simulink model "helicopter"  (R2020b)
settings: Solver=ode1  StartTime=0.0  StopTime=simulation_time  FixedStep=0.002  RelTol=1e-3  EnableMultiTasking=on
PostLoadFcn:
  | qc_set_target_type(getConfigSet(bdroot, 'QUARC Default Target Configuration'));
values from neighbouring files (symbols this model uses):
  elevation_gain = 1    [init.m]
  K_ed = 2*d_e*sqrt(K_ep/K_3)    [init.m]
  K_ei = K_ep*0.1    (= 0.348080190282)    [init.m]
  K_ep = w_e^2/K_3    (= 3.48080190282)    [init.m]
  K_pd = 2*d_p*sqrt(K_pp/K_1)    [init.m]
  K_pp = w_p^2/K_1    (= 5.8991559633)    [init.m]
  travel_gain = 1    [init.m]
  Vd_ff = V_d_eq    (= 0.1)    [init.m]
  Vs_ff = V_s_eq    (= 7.88)    [init.m]
  x1_0 = pi    (= 3.14159265359)    [problem_2.m]    (also in problem_4.m)
undefined symbols (not defined in the file or in its folder): HIL, K, qc_get_step_size
libraries: simulink_extras x9, quarc_library x4
settings Model: SimulationMode=external  ExtModeTrigDuration=5000  Creator=Rchan  LastModifiedBy=theodokl
settings SolverCC: PositivePriorityOrder=on
settings DataIOCC: SaveFormat=Array  SignalLoggingSaveFormat=ModelDataLogs  ReturnWorkspaceOutputs=off
settings OptimizationCC: ExpressionDepthLimit=2147483647  InitFltsAndDblsToZero=on  LifeSpan=inf
settings DebuggingCC: SaveWithParameterizedLinksMsg=none  UnderspecifiedInitializationDetection=Classic  MergeDetectMultiDrivingBlocksExec=none  SolverPrmCheckMsg=warning  MultiTaskDSMMsg=warning  MultiTaskCondExecSysMsg=none  FcnCallInpInsideContextMsg=warning  AllowSymbolicDim=off  StateNameClashWarn=warning  SFUnexpectedBacktrackingDiag=warning  SFNoUnconditionalDefaultTransitionDiag=warning  SFExecutionAtInitializationDiag=none  ArithmeticOperatorsInVariantConditions=warning
settings HardwareCC: ProdBitPerPointer=32  ProdBitPerSizeT=32  ProdBitPerPtrDiffT=32  ProdLargestAtomicFloat=None  ProdIntDivRoundTo=Undefined  ProdEndianess=Unspecified  ProdWordSize=32  ProdHWDeviceType=32-bit Generic
settings ModelReferenceCC: PropagateSignalLabelsOutOfModel=off
settings SFSimCC: SimUseLocalCustomCode=off  CustomCodeUndefinedFunction=UseInterfaceOnly
settings RTWCC: Description=QUARC Win64 Target  SystemTargetFile=quarc_win64.tlc  TemplateMakefile=quarc_default_tmf  RTWUseLocalCustomCode=off
settings CodeAppCC: StateflowObjectComments=on
settings GRTTargetCC: TargetLangStandard=C89/C90 (ANSI)  ParMdlRefBuildCompliant=off  CompOptLevelCompliant=off  CombineOutputUpdateFcns=off  MatFileLogging=off  GRTInterface=on  UseToolchainInfoCompliant=off  ExtMode=on  ExtModeMexFile=quarc_comm
settings ConfigComp: CovMetricSettings=dw  CovSaveCumulativeToWorkspaceVar=on  CovSaveSingleToWorkspaceVar=on  CovExternalEMLEnable=off  CovSFcnEnable=off

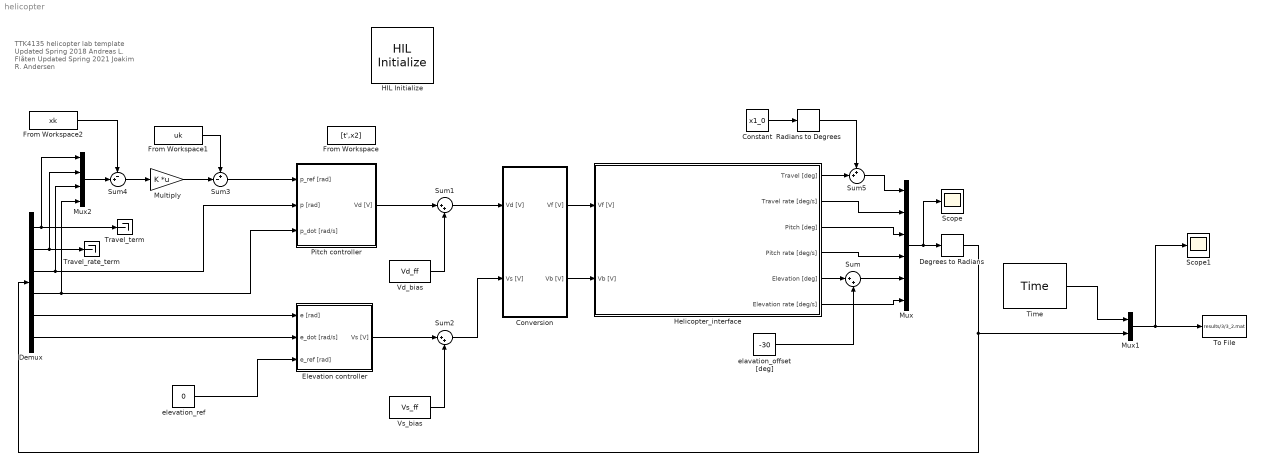
== system helicopter ==
  note: TTK4135 helicopter lab template
      | Updated Spring 2018
      | Andreas L. Flåten
      |
      | Updated Spring 2021
      | Joakim R. Andersen
  Constant : Constant  Value=x1_0
  Conversion : Subsystem
  Degrees to Radians : simulink_extras/Transformations/Degrees to Radians
  Demux : Demux  Outputs=6
  Elevation controller : Subsystem
  From Workspace : FromWorkspace  VariableName=[t',x2]  SampleTime=-1  OutputAfterFinalValue=Holding final value
  From Workspace1 : FromWorkspace  VariableName=uk
  From Workspace2 : FromWorkspace  VariableName=xk
  HIL Initialize : quarc_library/Data Acquisition/Generic/Configuration/HIL Initialize  Priority=-99  object_name=HIL-1  board_type=q8_usb  board_number=0  board_options=update_rate=normal;decimation=1  exclusive=off  active=off  hardware_clocks=[0:2]  clock_modes=[]  initial_clock_frequencies=[]  set_clock_params_at_start=off  set_clock_params_at_switch_in=off  set_clock_frequencies_at_start=off  set_clock_frequencies_at_switch_in=off  analog_input_channels=[0:7]  analog_input_configurations=[]  analog_input_maximums=10  analog_input_minimums=-10  set_analog_input_params_at_start=on  set_analog_input_params_at_switch_in=off  analog_output_channels=[0:7]  analog_output_maximums=10  analog_output_minimums=-10  initial_analog_outputs=[0]  final_analog_outputs=[0]  watchdog_analog_outputs=0  set_analog_output_params_at_start=on  set_analog_output_params_at_switch_in=off  set_analog_outputs_at_start=on  set_analog_outputs_at_switch_in=off  set_analog_outputs_at_terminate=on  set_analog_outputs_at_switch_out=off  set_analog_outputs_on_watchdog=off  digital_input_channels=[]  digital_output_channels=[]  digital_output_configuration=[]  initial_digital_outputs=[1]  final_digital_outputs=[1]  watchdog_digital_outputs=[1]  set_digital_output_params_at_start=off  set_digital_output_params_at_switch_in=off  set_digital_outputs_at_start=on  set_digital_outputs_at_switch_in=off  set_digital_outputs_at_terminate=on  set_digital_outputs_at_switch_out=off  set_digital_outputs_on_watchdog=off  encoder_channels=[0:7]  quadrature=[4]  encoder_filter_frequency=[]  initial_encoder_counts=[0]  set_encoder_params_at_start=on  set_encoder_params_at_switch_in=off  set_encoder_counts_at_start=on  set_encoder_counts_at_switch_in=off  pwm_channels=[0:7]  pwm_modes=0  pwm_frequency=99.532799999999995e6/4095  pwm_configuration=[0]  pwm_alignment=[0]  pwm_polarity=[1]  pwm_leading_deadband=[0]  pwm_trailing_deadband=[0]  initial_pwm_outputs=[0]  final_pwm_outputs=[0]  watchdog_pwm_outputs=[0]  set_pwm_params_at_start=on  set_pwm_params_at_switch_in=off  set_pwm_outputs_at_start=on  set_pwm_outputs_at_switch_in=off  set_pwm_outputs_at_terminate=on  set_pwm_outputs_at_switch_out=off  set_pwm_outputs_on_watchdog=off  other_output_channels=[]  initial_other_outputs=[]  final_other_outputs=[]  watchdog_other_outputs=[]  set_other_outputs_at_start=off  set_other_outputs_at_switch_in=off  set_other_outputs_at_terminate=off  set_other_outputs_at_switch_out=off  set_other_outputs_on_watchdog=off
  Helicopter_interface : Subsystem
  Multiply : Gain  Gain=K  Multiplication=Matrix(K*u)
  Mux : Mux  Inputs=6
  Mux1 : Mux  Inputs=2
  Mux2 : Mux
  Pitch controller : Subsystem
  Radians to Degrees : simulink_extras/Transformations/Radians to Degrees
  Scope : Scope
  Scope1 : Scope
  Sum : Sum  Inputs=|++
  Sum1 : Sum  Inputs=|++
  Sum2 : Sum  Inputs=|++
  Sum3 : Sum  Inputs=+-|
  Sum4 : Sum  Inputs=-+|
  Sum5 : Sum  Inputs=++|
  Time : quarc_library/Sources/Time/Time  time_source=Wall clock  sample_time=qc_get_step_size
  To File : ToFile  Filename=results/3/3_2.mat  MatrixName=simout
  Travel_rate_term : Terminator
  Travel_term : Terminator
  Vd_bias : Constant  Value=Vd_ff
  Vs_bias : Constant  Value=Vs_ff
  elavation_offset [deg] : Constant  Value=-30
  elevation_ref : Constant  Value=0
  wires:
  Conversion/2(Vb [V]) -> Helicopter_interface/2(Vb [V])
  Conversion/1(Vf [V]) -> Helicopter_interface/1(Vf [V])
  elavation_offset [deg]/1 -> Sum/2
  Helicopter_interface/5(Elevation [deg]) -> Sum/1
  Helicopter_interface/4(Pitch rate [deg/s]) -> Mux/4
  Helicopter_interface/3(Pitch [deg]) -> Mux/3
  Helicopter_interface/2(Travel rate [deg/s]) -> Mux/2
  Sum/1 -> Mux/5
  Helicopter_interface/6(Elevation rate [deg/s]) -> Mux/6
  Mux/1 -> Scope/1, Degrees to Radians/1
  Degrees to Radians/1 -> Mux1/2, Demux/1
  Demux/1 -> Mux2/1, Travel_term/1
  Demux/2 -> Mux2/2, Travel_rate_term/1
  Demux/3 -> Mux2/3, Pitch controller/2(p [rad])
  Demux/4 -> Pitch controller/3(p_dot [rad/s]), Mux2/4
  Demux/6 -> Elevation controller/2(e_dot [rad/s])
  Demux/5 -> Elevation controller/1(e [rad])
  elevation_ref/1 -> Elevation controller/3(e_ref [rad])
  Vd_bias/1 -> Sum1/2
  Pitch controller/1(Vd [V]) -> Sum1/1
  Vs_bias/1 -> Sum2/2
  Elevation controller/1(Vs [V]) -> Sum2/1
  Mux1/1 -> To File/1, Scope1/1
  Sum1/1 -> Conversion/1(Vd [V])
  Sum2/1 -> Conversion/2(Vs [V])
  Time/1 -> Mux1/1
  Sum3/1 -> Pitch controller/1(p_ref [rad])
  From Workspace1/1 -> Sum3/1
  Multiply/1 -> Sum3/2
  Sum4/1 -> Multiply/1
  From Workspace2/1 -> Sum4/1
  Mux2/1 -> Sum4/2
  Helicopter_interface/1(Travel [deg]) -> Sum5/2
  Sum5/1 -> Mux/1
  Radians to Degrees/1 -> Sum5/1
  Constant/1 -> Radians to Degrees/1

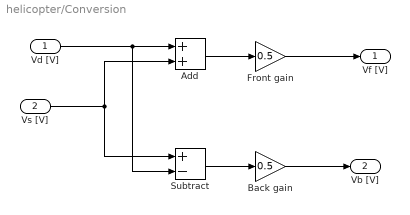
== system helicopter/Conversion ==
  Vd [V] : Inport
  Vs [V] : Inport  Port=2
  Add : Sum
  Back gain : Gain  Gain=0.5
  Front gain : Gain  Gain=0.5
  Subtract : Sum  Inputs=+-
  Vf [V] : Outport
  Vb [V] : Outport  Port=2
  wires:
  Vd [V]/1 -> Subtract/2, Add/1
  Vs [V]/1 -> Subtract/1, Add/2
  Subtract/1 -> Back gain/1
  Back gain/1 -> Vb [V]/1
  Add/1 -> Front gain/1
  Front gain/1 -> Vf [V]/1

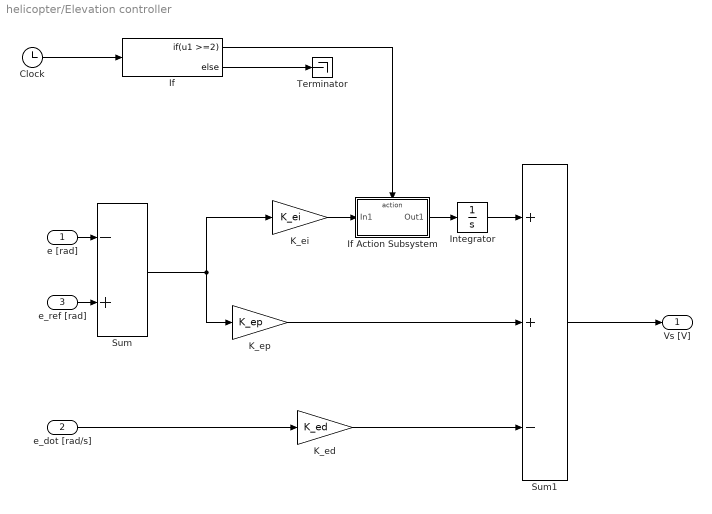
== system helicopter/Elevation controller ==
  e [rad] : Inport
  e_dot [rad/s] : Inport  Port=2
  e_ref [rad] : Inport  Port=3
  Clock : Clock
  If : If  IfExpression=u1 >=2
  If Action Subsystem : Subsystem  TreatAsAtomicUnit=on
  Integrator : Integrator  LimitOutput=on
  K_ed : Gain  Gain=K_ed  SaturateOnIntegerOverflow=on  OutDataTypeStr=Inherit: Same as input  ParamDataTypeStr=Inherit: Same as input
  K_ei : Gain  Gain=K_ei  SaturateOnIntegerOverflow=on  OutDataTypeStr=Inherit: Same as input  ParamDataTypeStr=Inherit: Same as input
  K_ep : Gain  Gain=K_ep  SaturateOnIntegerOverflow=on  OutDataTypeStr=Inherit: Same as input  ParamDataTypeStr=Inherit: Same as input
  Sum : Sum  Inputs=-+  InputSameDT=on  SaturateOnIntegerOverflow=on  OutDataTypeStr=Inherit: Same as first input
  Sum1 : Sum  Inputs=++-  InputSameDT=on  SaturateOnIntegerOverflow=on  OutDataTypeStr=Inherit: Same as first input
  Terminator : Terminator
  Vs [V] : Outport  InitialOutput=0
  wires:
  K_ed/1 -> Sum1/3
  e_dot [rad/s]/1 -> K_ed/1
  Sum1/1 -> Vs [V]/1
  K_ei/1 -> If Action Subsystem/1(In1)
  If Action Subsystem/1(Out1) -> Integrator/1
  If/2 -> Terminator/1
  Clock/1 -> If/1
  e [rad]/1 -> Sum/1
  K_ep/1 -> Sum1/2
  e_ref [rad]/1 -> Sum/2
  Sum/1 -> K_ep/1, K_ei/1
  If/1 -> If Action Subsystem/Action
  Integrator/1 -> Sum1/1

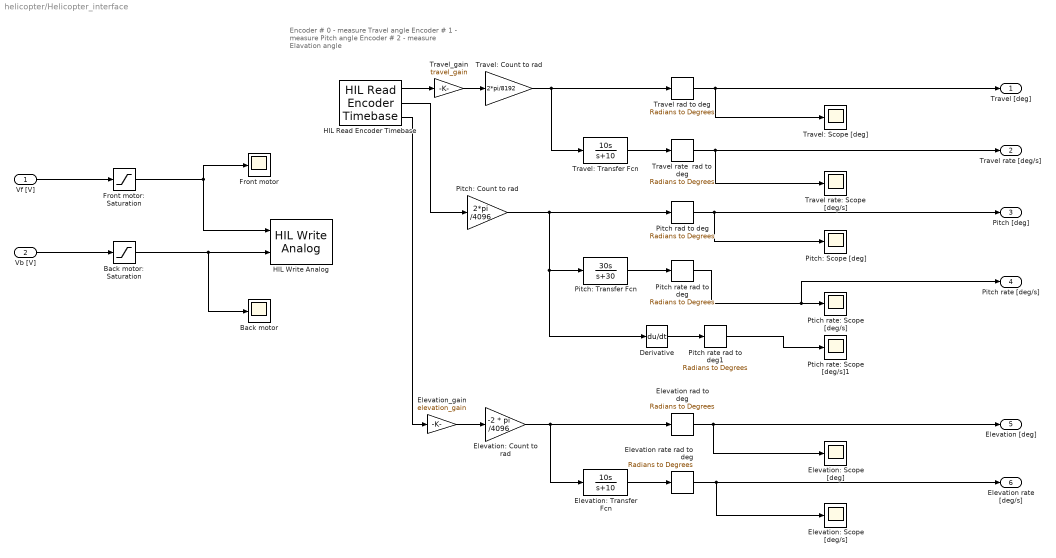
== system helicopter/Helicopter_interface ==
  note: Encoder # 0 - measure Travel angle
      | Encoder # 1 - measure Pitch angle
      | Encoder # 2 - measure Elavation angle
  Vf [V] : Inport
  Vb [V] : Inport  Port=2
  Back motor : Scope
  Back motor: Saturation : Saturate  UpperLimit=5  LowerLimit=-5
  Derivative : Derivative
  Elevation rad to deg : simulink_extras/Transformations/Radians to Degrees
  Elevation rate rad to deg : simulink_extras/Transformations/Radians to Degrees
  Elevation: Count to rad : Gain  Gain=-2 * pi /4096
  Elevation: Scope [deg/s] : Scope
  Elevation: Scope [deg] : Scope
  Elevation: Transfer Fcn : TransferFcn  Numerator=[10 0]  Denominator=[1 10]
  Elevation_gain : Gain  Gain=elevation_gain
  Front motor : Scope
  Front motor: Saturation : Saturate  UpperLimit=5  LowerLimit=-5
  HIL Read Encoder Timebase : quarc_library/Data Acquisition/Generic/Timebases/HIL Read Encoder Timebase  object_name=HIL-1  clock=0  channels=[0:2]  active=on  vector_output=off  data_type_mode=Inherit via back propagation  data_type=double  overflow_mode=Error on overflow  samples_in_buffer=max(ceil(1/qc_get_step_size), 1)
  HIL Write Analog : quarc_library/Data Acquisition/Generic/Immediate I//O/HIL Write Analog  object_name=HIL-1  channels=[0:1]  sample_time=-1  active=off  vector_input=off
  Pitch rad to deg : simulink_extras/Transformations/Radians to Degrees
  Pitch rate rad to deg : simulink_extras/Transformations/Radians to Degrees
  Pitch rate rad to deg1 : simulink_extras/Transformations/Radians to Degrees
  Pitch: Count to rad : Gain  Gain=2*pi /4096
  Pitch: Scope [deg] : Scope
  Pitch: Transfer Fcn : TransferFcn  Numerator=[30 0]  Denominator=[1 30]
  Ptich rate: Scope [deg/s] : Scope
  Ptich rate: Scope [deg/s]1 : Scope
  Travel rad to deg : simulink_extras/Transformations/Radians to Degrees
  Travel rate  rad to deg : simulink_extras/Transformations/Radians to Degrees
  Travel rate: Scope [deg/s] : Scope
  Travel: Count to rad : Gain  Gain=2*pi/8192
  Travel: Scope [deg] : Scope
  Travel: Transfer Fcn : TransferFcn  Numerator=[10 0]  Denominator=[1 10]
  Travel_gain : Gain  Gain=travel_gain
  Travel [deg] : Outport
  Travel rate [deg/s] : Outport  Port=2
  Pitch [deg] : Outport  Port=3
  Pitch rate [deg/s] : Outport  Port=4
  Elevation [deg] : Outport  Port=5
  Elevation rate [deg/s] : Outport  Port=6
  wires:
  HIL Read Encoder Timebase/1 -> Travel_gain/1
  HIL Read Encoder Timebase/2 -> Pitch: Count to rad/1
  HIL Read Encoder Timebase/3 -> Elevation_gain/1
  Travel: Count to rad/1 -> Travel: Transfer Fcn/1, Travel rad to deg/1
  Travel: Transfer Fcn/1 -> Travel rate  rad to deg/1
  Pitch: Transfer Fcn/1 -> Pitch rate rad to deg/1
  Elevation: Count to rad/1 -> Elevation: Transfer Fcn/1, Elevation rad to deg/1
  Elevation: Transfer Fcn/1 -> Elevation rate rad to deg/1
  Travel rad to deg/1 -> Travel: Scope [deg]/1, Travel [deg]/1
  Travel rate  rad to deg/1 -> Travel rate: Scope [deg/s]/1, Travel rate [deg/s]/1
  Vf [V]/1 -> Front motor: Saturation/1
  Vb [V]/1 -> Back motor: Saturation/1
  Front motor: Saturation/1 -> HIL Write Analog/1, Front motor/1
  Back motor: Saturation/1 -> Back motor/1, HIL Write Analog/2
  Derivative/1 -> Pitch rate rad to deg1/1
  Pitch: Count to rad/1 -> Derivative/1, Pitch: Transfer Fcn/1, Pitch rad to deg/1
  Pitch rate rad to deg1/1 -> Ptich rate: Scope [deg/s]1/1
  Pitch rad to deg/1 -> Pitch [deg]/1, Pitch: Scope [deg]/1
  Pitch rate rad to deg/1 -> Pitch rate [deg/s]/1, Ptich rate: Scope [deg/s]/1
  Elevation rad to deg/1 -> Elevation [deg]/1, Elevation: Scope [deg]/1
  Elevation rate rad to deg/1 -> Elevation rate [deg/s]/1, Elevation: Scope [deg/s]/1
  Travel_gain/1 -> Travel: Count to rad/1
  Elevation_gain/1 -> Elevation: Count to rad/1

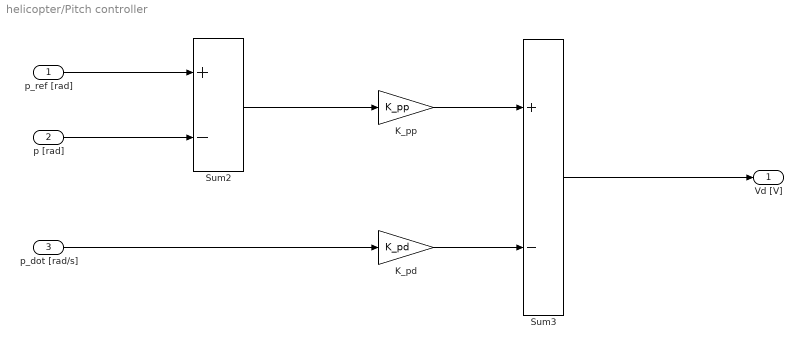
== system helicopter/Pitch controller ==
  p_ref [rad] : Inport
  p [rad] : Inport  Port=2
  p_dot [rad/s] : Inport  Port=3
  K_pd : Gain  Gain=K_pd  SaturateOnIntegerOverflow=on  OutDataTypeStr=Inherit: Same as input  ParamDataTypeStr=Inherit: Same as input
  K_pp : Gain  Gain=K_pp  SaturateOnIntegerOverflow=on  OutDataTypeStr=Inherit: Same as input  ParamDataTypeStr=Inherit: Same as input
  Sum2 : Sum  Inputs=+-  InputSameDT=on  SaturateOnIntegerOverflow=on  OutDataTypeStr=Inherit: Same as first input
  Sum3 : Sum  Inputs=+-  InputSameDT=on  SaturateOnIntegerOverflow=on  OutDataTypeStr=Inherit: Same as first input
  Vd [V] : Outport  InitialOutput=0
  wires:
  p_ref [rad]/1 -> Sum2/1
  p [rad]/1 -> Sum2/2
  p_dot [rad/s]/1 -> K_pd/1
  K_pp/1 -> Sum3/1
  Sum2/1 -> K_pp/1
  K_pd/1 -> Sum3/2
  Sum3/1 -> Vd [V]/1

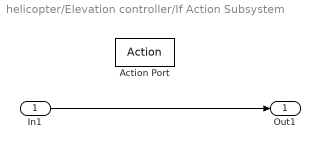
== system helicopter/Elevation controller/If Action Subsystem ==
  In1 : Inport
  Action Port : ActionPort  ActionPortLabel=if(u1 >=2)
  Out1 : Outport
  wires:
  In1/1 -> Out1/1
